simulink model "gmp_pmsm_sensored_nonlinear_sil_mdl_2022b"  (R2022b)
settings: Solver=VariableStepAuto  StartTime=0.0  StopTime=10  RelTol=1e-3
model workspace (MAT data in the model file):
  B = 0
  BW_i = 800
  Flux_t = 0.12
  IQ24 : Simulink.NumericType (value not decoded)
  J = 0.018
  K_d = 3.72061852168
  K_m = 0.128242020589
  K_u = 0.00236407598332
  Ki_id = 0.001
  Ki_iq = 1
  Ki_n = 25225.1136556
  Kp_id = 1e-05
  Kp_iq = 5e-05
  Kp_n = 12.6125568278
  Ld_t = 0.00303
  Lq_t = 0.02019
  Max_p = 0.006000830667
  P = 2
  RLS_ini_a = 1000000
  Rd_mos = 0.01
  Rs = 0.1215
  Rv = 6.4
  T_final = 0
  T_initial = 0
  Tes = [4 7 10 7 4]
  Tf_t = 0.1
  Tm = 0
  Udq_limit = 550
  Var = 0
  Vce0 = 0
  Vd0 = 0
  Vdc = 80
  button = 1
  im_limit = 40
  mean_prd = 10
  position_init = 0.2
  r_ce = 1e-08
  r_d = 1e-08
  sample_prd = 100
  step_time = 0.2
  ts = 6.25e-05
  wc = 3500
libraries: peripheral_utilities x9, spsSeriesRLCBranchLib x6, spsMosfetLib x6, simulink x3, spsVoltageMeasurementLib x2, gmp_sil_core_pack x1, spsPermanentMagnetSynchronousMachineLib x1, spsdq0toabcLib x1, spsFourierLib x1, spsControlledVoltageSourceLib x1, sps_lib x1
(part 3 of 3)

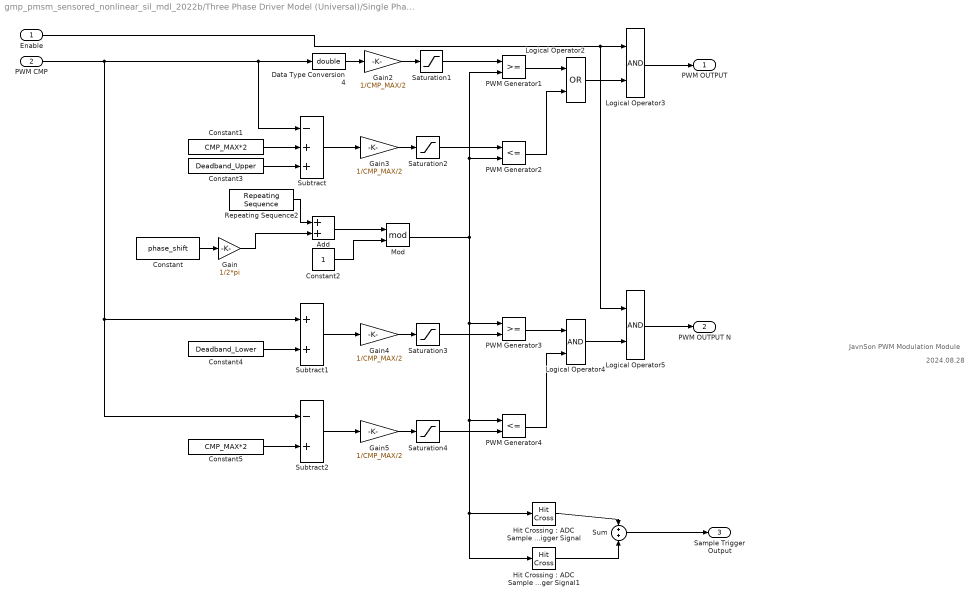
== system gmp_pmsm_sensored_nonlinear_sil_mdl_2022b/Three Phase Driver Model (Universal)/Single Phase Full Bridge V/Triangle PWM modulation (with deadband)1 ==
  note: JavnSon PWM Modulation Module
  note: 2024.08.28
  Enable : Inport
  PWM CMP : Inport  Port=2
  Add : Sum
  Constant : Constant  Value=phase_shift
  Constant1 : Constant  Value=CMP_MAX*2
  Constant2 : Constant
  Constant3 : Constant  Value=Deadband_Upper
  Constant4 : Constant  Value=Deadband_Lower
  Constant5 : Constant  Value=CMP_MAX*2
  Data Type Conversion4 : DataTypeConversion  OutDataTypeStr=double  SaturateOnIntegerOverflow=off  RndMeth=Floor
  Gain : Gain  Gain=1/2*pi
  Gain{2..5} (4 alike) : Gain  Gain=1/CMP_MAX/2
  Hit Crossing：ADC Sample Trigger Signal : HitCross  HitCrossingOffset=0.5  HitCrossingDirection=rising
  Hit Crossing：ADC Sample Trigger Signal1 : HitCross  HitCrossingOffset=0.5  HitCrossingDirection=falling
  Logical Operator2 : Logic  Operator=OR  AllPortsSameDT=off  OutDataTypeStr=boolean
  Logical Operator3 : Logic  AllPortsSameDT=off  OutDataTypeStr=boolean
  Logical Operator4 : Logic  AllPortsSameDT=off  OutDataTypeStr=boolean
  Logical Operator5 : Logic  AllPortsSameDT=off  OutDataTypeStr=boolean
  Mod : Math  Operator=mod
  PWM Generator1 : RelationalOperator  OutDataTypeStr=boolean  InputSameDT=off
  PWM Generator2 : RelationalOperator  Operator=<=  OutDataTypeStr=boolean  InputSameDT=off
  PWM Generator3 : RelationalOperator  OutDataTypeStr=boolean  InputSameDT=off
  PWM Generator4 : RelationalOperator  Operator=<=  OutDataTypeStr=boolean  InputSameDT=off
  Repeating Sequence2 : simulink/Sources/Repeating Sequence  rep_seq_t=[0, 1/2/fswitch, 1/fswitch ]  rep_seq_y=[0,0.5,1]
  Saturation{1..4} (4 alike) : Saturate  UpperLimit=1  LowerLimit=0
  Subtract : Sum  Inputs=-++
  Subtract1 : Sum
  Subtract2 : Sum  Inputs=-+
  Sum : Sum  Inputs=+|+
  PWM OUTPUT : Outport
  PWM OUTPUT N : Outport  Port=2
  Sample Trigger Output : Outport  Port=3
  wires:
  Constant/1 -> Gain/1
  Constant2/1 -> Mod/2
  Add/1 -> Mod/1
  Gain/1 -> Add/2
  Repeating Sequence2/1 -> Add/1
  Logical Operator3/1 -> PWM OUTPUT/1
  Logical Operator5/1 -> PWM OUTPUT N/1
  Enable/1 -> Logical Operator3/1, Logical Operator5/1
  Mod/1 -> PWM Generator4/1, Hit Crossing：ADC Sample Trigger Signal1/1, Hit Crossing：ADC Sample Trigger Signal/1, PWM Generator3/1, PWM Generator1/2, PWM Generator2/2
  Logical Operator4/1 -> Logical Operator5/2
  PWM Generator4/1 -> Logical Operator4/2
  Subtract2/1 -> Gain5/1
  Gain5/1 -> Saturation4/1
  Saturation4/1 -> PWM Generator4/2
  Constant5/1 -> Subtract2/2
  PWM Generator3/1 -> Logical Operator4/1
  Saturation3/1 -> PWM Generator3/2
  Subtract1/1 -> Gain4/1
  Gain4/1 -> Saturation3/1
  Constant4/1 -> Subtract1/2
  Saturation2/1 -> PWM Generator2/1
  Subtract/1 -> Gain3/1
  Gain3/1 -> Saturation2/1
  PWM Generator2/1 -> Logical Operator2/2
  Constant3/1 -> Subtract/3
  Constant1/1 -> Subtract/2
  Logical Operator2/1 -> Logical Operator3/2
  PWM Generator1/1 -> Logical Operator2/1
  Saturation1/1 -> PWM Generator1/1
  Gain2/1 -> Saturation1/1
  Data Type Conversion4/1 -> Gain2/1
  PWM CMP/1 -> Data Type Conversion4/1, Subtract/1, Subtract1/1, Subtract2/1
  Sum/1 -> Sample Trigger Output/1
  Hit Crossing：ADC Sample Trigger Signal/1 -> Sum/1
  Hit Crossing：ADC Sample Trigger Signal1/1 -> Sum/2

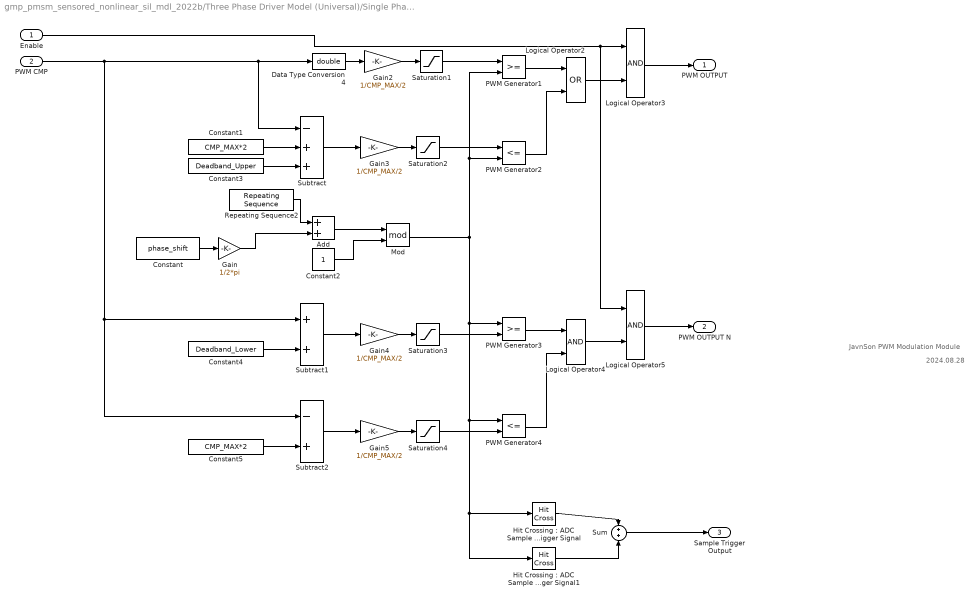
== system gmp_pmsm_sensored_nonlinear_sil_mdl_2022b/Three Phase Driver Model (Universal)/Single Phase Full Bridge W/Triangle PWM modulation (with deadband)1 ==
  note: JavnSon PWM Modulation Module
  note: 2024.08.28
  Enable : Inport
  PWM CMP : Inport  Port=2
  Add : Sum
  Constant : Constant  Value=phase_shift
  Constant1 : Constant  Value=CMP_MAX*2
  Constant2 : Constant
  Constant3 : Constant  Value=Deadband_Upper
  Constant4 : Constant  Value=Deadband_Lower
  Constant5 : Constant  Value=CMP_MAX*2
  Data Type Conversion4 : DataTypeConversion  OutDataTypeStr=double  SaturateOnIntegerOverflow=off  RndMeth=Floor
  Gain : Gain  Gain=1/2*pi
  Gain{2..5} (4 alike) : Gain  Gain=1/CMP_MAX/2
  Hit Crossing：ADC Sample Trigger Signal : HitCross  HitCrossingOffset=0.5  HitCrossingDirection=rising
  Hit Crossing：ADC Sample Trigger Signal1 : HitCross  HitCrossingOffset=0.5  HitCrossingDirection=falling
  Logical Operator2 : Logic  Operator=OR  AllPortsSameDT=off  OutDataTypeStr=boolean
  Logical Operator3 : Logic  AllPortsSameDT=off  OutDataTypeStr=boolean
  Logical Operator4 : Logic  AllPortsSameDT=off  OutDataTypeStr=boolean
  Logical Operator5 : Logic  AllPortsSameDT=off  OutDataTypeStr=boolean
  Mod : Math  Operator=mod
  PWM Generator1 : RelationalOperator  OutDataTypeStr=boolean  InputSameDT=off
  PWM Generator2 : RelationalOperator  Operator=<=  OutDataTypeStr=boolean  InputSameDT=off
  PWM Generator3 : RelationalOperator  OutDataTypeStr=boolean  InputSameDT=off
  PWM Generator4 : RelationalOperator  Operator=<=  OutDataTypeStr=boolean  InputSameDT=off
  Repeating Sequence2 : simulink/Sources/Repeating Sequence  rep_seq_t=[0, 1/2/fswitch, 1/fswitch ]  rep_seq_y=[0,0.5,1]
  Saturation{1..4} (4 alike) : Saturate  UpperLimit=1  LowerLimit=0
  Subtract : Sum  Inputs=-++
  Subtract1 : Sum
  Subtract2 : Sum  Inputs=-+
  Sum : Sum  Inputs=+|+
  PWM OUTPUT : Outport
  PWM OUTPUT N : Outport  Port=2
  Sample Trigger Output : Outport  Port=3
  wires:
  Constant/1 -> Gain/1
  Constant2/1 -> Mod/2
  Add/1 -> Mod/1
  Gain/1 -> Add/2
  Repeating Sequence2/1 -> Add/1
  Logical Operator3/1 -> PWM OUTPUT/1
  Logical Operator5/1 -> PWM OUTPUT N/1
  Enable/1 -> Logical Operator3/1, Logical Operator5/1
  Mod/1 -> PWM Generator4/1, Hit Crossing：ADC Sample Trigger Signal1/1, Hit Crossing：ADC Sample Trigger Signal/1, PWM Generator3/1, PWM Generator1/2, PWM Generator2/2
  Logical Operator4/1 -> Logical Operator5/2
  PWM Generator4/1 -> Logical Operator4/2
  Subtract2/1 -> Gain5/1
  Gain5/1 -> Saturation4/1
  Saturation4/1 -> PWM Generator4/2
  Constant5/1 -> Subtract2/2
  PWM Generator3/1 -> Logical Operator4/1
  Saturation3/1 -> PWM Generator3/2
  Subtract1/1 -> Gain4/1
  Gain4/1 -> Saturation3/1
  Constant4/1 -> Subtract1/2
  Saturation2/1 -> PWM Generator2/1
  Subtract/1 -> Gain3/1
  Gain3/1 -> Saturation2/1
  PWM Generator2/1 -> Logical Operator2/2
  Constant3/1 -> Subtract/3
  Constant1/1 -> Subtract/2
  Logical Operator2/1 -> Logical Operator3/2
  PWM Generator1/1 -> Logical Operator2/1
  Saturation1/1 -> PWM Generator1/1
  Gain2/1 -> Saturation1/1
  Data Type Conversion4/1 -> Gain2/1
  PWM CMP/1 -> Data Type Conversion4/1, Subtract/1, Subtract1/1, Subtract2/1
  Sum/1 -> Sample Trigger Output/1
  Hit Crossing：ADC Sample Trigger Signal/1 -> Sum/1
  Hit Crossing：ADC Sample Trigger Signal1/1 -> Sum/2

== system gmp_pmsm_sensored_nonlinear_sil_mdl_2022b/SynRM1/Electrical model/Subsystem/Angle converter ==
  theta : Inport
  Gain : Gain  Gain=180/pi
  Trigonometric Function : Trigonometry
  Trigonometric Function1 : Trigonometry  Operator=cos
  Trigonometric Function2 : Trigonometry  Operator=atan2
  the_deg : Outport  VectorParamsAs1DForOutWhenUnconnected=off
  wires:
  Trigonometric Function1/1 -> Trigonometric Function2/2
  Gain/1 -> the_deg/1
  Trigonometric Function2/1 -> Gain/1
  Trigonometric Function/1 -> Trigonometric Function2/1
  theta/1 -> Trigonometric Function1/1, Trigonometric Function/1

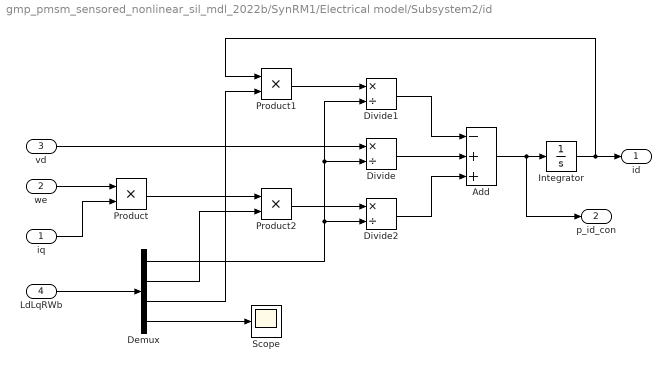
== system gmp_pmsm_sensored_nonlinear_sil_mdl_2022b/SynRM1/Electrical model/Subsystem2/id ==
  iq : Inport
  we : Inport  Port=2
  vd : Inport  Port=3
  LdLqRWb : Inport  Port=4
  Add : Sum  Inputs=-++
  Demux : Demux
  Divide : Product  Inputs=*/
  Divide1 : Product  Inputs=*/
  Divide2 : Product  Inputs=*/
  Integrator : Integrator
  Product : Product
  Product1 : Product
  Product2 : Product
  Scope : Scope
  id : Outport  VectorParamsAs1DForOutWhenUnconnected=off
  p_id_con : Outport  Port=2
  wires:
  we/1 -> Product/1
  iq/1 -> Product/2
  LdLqRWb/1 -> Demux/1
  Product/1 -> Product2/1
  Demux/2 -> Product2/2
  Demux/1 -> Divide1/2, Divide/2, Divide2/2
  Product2/1 -> Divide2/1
  vd/1 -> Divide/1
  Demux/3 -> Product1/2
  Integrator/1 -> Product1/1, id/1
  Add/1 -> p_id_con/1, Integrator/1
  Product1/1 -> Divide1/1
  Divide1/1 -> Add/1
  Divide/1 -> Add/2
  Divide2/1 -> Add/3
  Demux/4 -> Scope/1

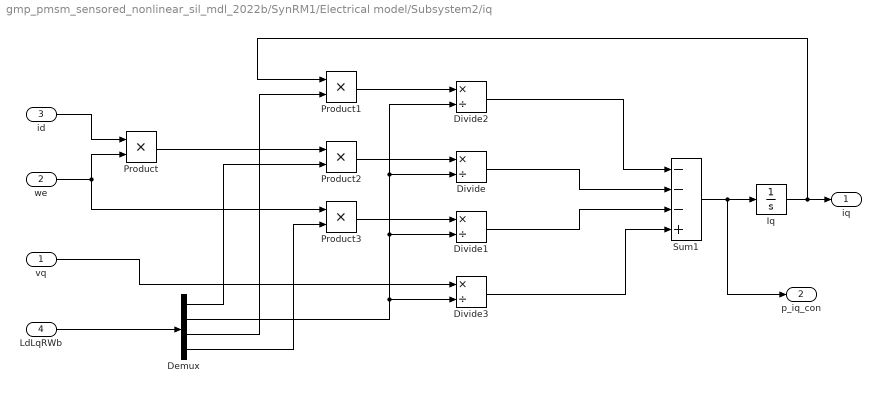
== system gmp_pmsm_sensored_nonlinear_sil_mdl_2022b/SynRM1/Electrical model/Subsystem2/iq ==
  vq : Inport
  we : Inport  Port=2
  id : Inport  Port=3
  LdLqRWb : Inport  Port=4
  Demux : Demux
  Divide{,1..3} (4 alike) : Product  Inputs=*/
  Iq : Integrator
  Product{,1..3} (4 alike) : Product
  Sum1 : Sum  Inputs=---+
  iq : Outport  VectorParamsAs1DForOutWhenUnconnected=off
  p_iq_con : Outport  Port=2
  wires:
  LdLqRWb/1 -> Demux/1
  Sum1/1 -> p_iq_con/1, Iq/1
  Iq/1 -> Product1/1, iq/1
  we/1 -> Product3/1, Product/2
  id/1 -> Product/1
  Demux/2 -> Divide1/2, Divide2/2, Divide/2, Divide3/2
  Product1/1 -> Divide2/1
  Demux/3 -> Product1/2
  Demux/1 -> Product2/2
  Product/1 -> Product2/1
  Demux/4 -> Product3/2
  vq/1 -> Divide3/1
  Divide2/1 -> Sum1/1
  Divide/1 -> Sum1/2
  Product2/1 -> Divide/1
  Product3/1 -> Divide1/1
  Divide1/1 -> Sum1/3
  Divide3/1 -> Sum1/4
